simulink model "Links_TCP_Demo"  (R2022b)
settings: Solver=FixedStepAuto  StartTime=0.0  StopTime=inf  FixedStep=0.001  RelTol=1e-3
libraries: Links_TCP_Lib x6
settings Model: Creator=lwc  LastModifiedBy=Administrator
settings SolverCC: AlgebraicLoopSolver=TrustRegion
settings DataIOCC: ReturnWorkspaceOutputs=off
settings DebuggingCC: UnconnectedInputMsg=warning  UnconnectedOutputMsg=warning  UnconnectedLineMsg=warning  SFMachineParentedDataDiag=warning  ArithmeticOperatorsInVariantConditions=warning
settings HardwareCC: ProdBitPerLong=64  ProdHWDeviceType=Intel->x86-64 (Linux 64)
settings ModelReferenceCC: EnableRefExpFcnMdlSchedulingChecks=on
settings SFSimCC: SimUseLocalCustomCode=off  CustomCodeUndefinedFunction=UseInterfaceOnly
settings RTWCC: SystemTargetFile=links_rtlnx_grt.tlc  TemplateMakefile=links_rtlnx_grt.tmf  RTWUseLocalCustomCode=off
settings CodeAppCC: StateflowObjectComments=on
settings STFCustomTargetCC: TargetLangStandard=C99 (ISO)  CombineOutputUpdateFcns=on  SystemTargetFile=links_rtlnx_grt.tlc
settings GRTTargetCC: ParMdlRefBuildCompliant=off  CompOptLevelCompliant=off  ConcurrentExecutionCompliant=off  MatFileLogging=off  CPPClassGenCompliant=off  UseToolchainInfoCompliant=off  RTWCAPISignals=on  RTWCAPIParams=on  RTWCAPIRootIO=on

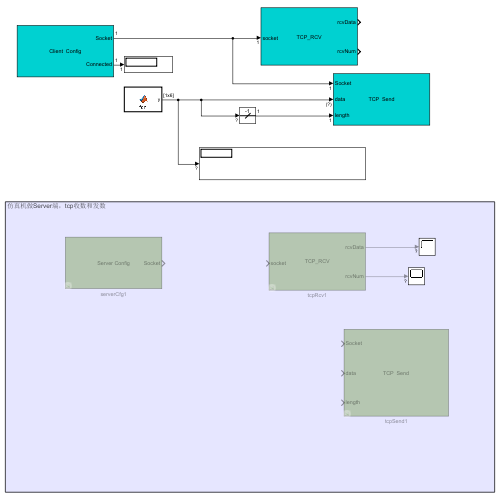
[thumbnail: Simulink's stored preview of the top-level diagram]
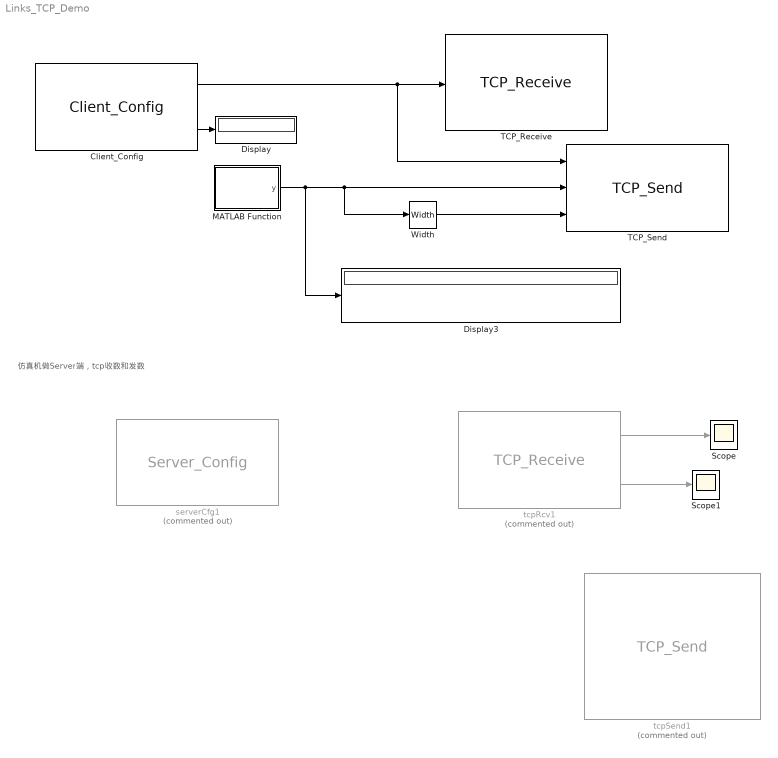
== system Links_TCP_Demo ==
  note: 仿真机做Server端，tcp收数和发数
  Client_Config : Links_TCP_Lib/Client_Config  serverIp=192.168.1.220  serverPort=5025  sampleTime=-1
      settings: SourceProductName=Links_LnxLib
  Display : Display
  Display3 : Display
      settings: Format=hex (Stored Integer)
  MATLAB Function : MATLAB Function  TreatAsAtomicUnit=on
  Scope : Scope
  Scope1 : Scope
  TCP_Receive : Links_TCP_Lib/TCP_Receive  width=128  sampletime=-1
      settings: SourceProductName=Links_LnxLib
  TCP_Send : Links_TCP_Lib/TCP_Send  sampleTime=-1
      settings: SourceProductName=Links_LnxLib
  Width : Width  DataType=int32
  serverCfg1 : Links_TCP_Lib/Server_Config  Commented=on  serverIp=192.168.1.220  serverPort=5025  clientNum=1  clientIp=192.168.1.240  sampleTime=-1
      settings: SourceProductName=Links_LnxLib
  tcpRcv1 : Links_TCP_Lib/TCP_Receive  Commented=on  width=20  sampletime=1
      settings: SourceProductName=Links_LnxLib
  tcpSend1 : Links_TCP_Lib/TCP_Send  Commented=on  sampleTime=-1
      settings: SourceProductName=Links_LnxLib
  wires:
  Width/1 -> TCP_Send/3
  tcpRcv1/2 -> Scope1/1
  tcpRcv1/1 -> Scope/1
  Client_Config/1 -> TCP_Send/1, TCP_Receive/1
  Client_Config/2 -> Display/1
  MATLAB Function/1(y) -> Display3/1, Width/1, TCP_Send/2

== matlab function Links_TCP_Demo/MATLAB Function ==
  data: y output
function y = fcn()

y = [uint8('*IDN?'),uint8(10)];
